simulink model "TB19_R2_Integrated_Shed"  (R2025a)
settings: Solver=FixedStepDiscrete  StartTime=0  StopTime=TB.t_end  FixedStep=TB.dt  RelTol=1e-3
InitFcn:
  | % 모델과 같은 폴더의 초기화 스크립트를 실행해 P(설계 파라미터)와 TB(시험 조건)를 만든다.
  | run(fullfile(fileparts(get_param(bdroot, 'FileName')), 'TB19_init.m'));
values from neighbouring files (symbols this model uses):
  TB = struct()    [TB19_init.m]    (also in run_TB19.m = evalin('base', 'TB'))
libraries: fl_lib x158, nesl_utility x67
(part 1 of 4)
settings Model: Creator=hj000  LastModifiedBy=hj000
settings DataIOCC: SaveOutput=off  SignalLogging=off  SaveTime=off

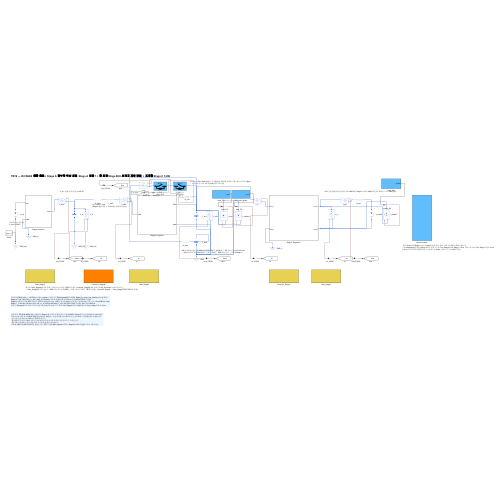
[thumbnail: Simulink's stored preview of the top-level diagram]
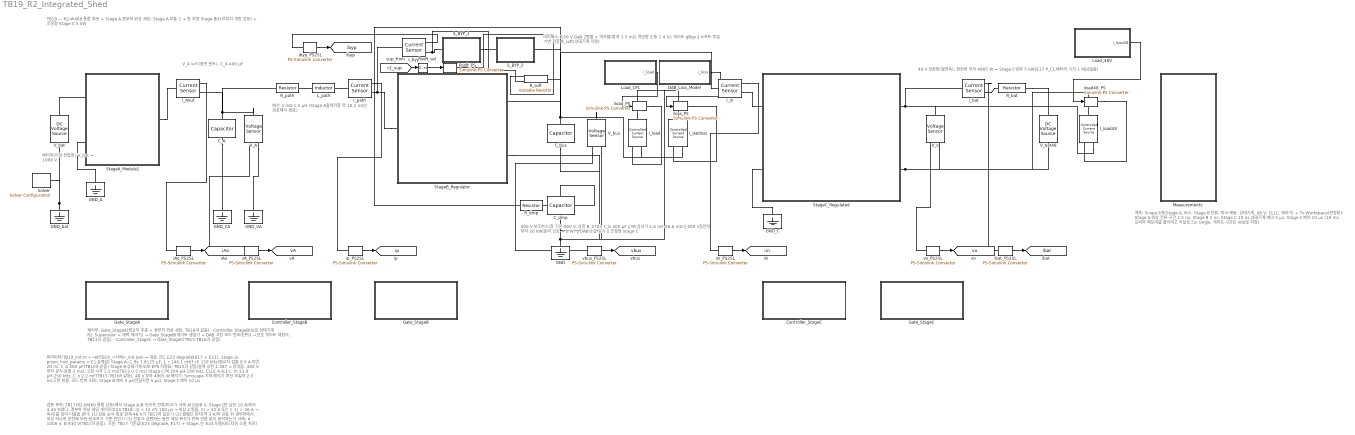
== system TB19_R2_Integrated_Shed ==
  note: TB19 — R2-W460 통합 회로 + Stage A 경부하 위상 셰딩: Stage A 모듈 1 + 창 조정 Stage B(H-브리지 개방 강등) + 조정형 Stage C 5 kW
  note: 배터리(이상 전압원)
      | V_bat = 1008 V
  note: V_A 노드(충전 포트), C_A 400 µF
  note: 배선 3 mΩ·1.5 µH
      | (Stage A 출력저항 약 10.2 mΩ는 회로에서 생김)
  note: 바이패스: 150 V GaN 2병렬 × 역직렬(합계 3.3 mΩ, 역방향 도통 1.4 V), 게이트 gByp
      | ∥ 소프트 투입 가변 저항 R_soft(상태기계 지령)
  note: 400 V 보조버스(창 기준 460 V, 상한 B_470): C_b 400 µF ∥ RC 감쇠기 1.6 mF·48.6 mΩ
      | ∥ 400 V 정전력 부하 20 kW(분리 신호 → 0 W) ∥ DAB 손실 등가 ∥ 조정형 Stage C
  note: 48 V 전원망(절연측): 정전력 부하 4905 W = Stage C 입력 5 kW(E17 P_C), 배터리 가지 1 MΩ(없음)
  note: 제어부: Gate_StageA(영교차 추종 + 경부하 위상 셰딩, TB18과 같음) · Controller_StageB(보호 상태기계 R2_Supervisor + 채택 제어기)
      | → Gate_StageB(게이트 생성기 + DAB 고장 모드 변조(EPS) → 보호 게이트 재정의, TB13과 같음) · Controller_StageC → Gate_StageC(TB15·TB16과 같음)
  note: 계측: Scope 8개(Stage A, 버스, Stage B 전류, 링크·제동, 상태기계, 48 V, CLLC, 제어기)
      | + To Workspace(판정용): Stage A 위상 전류·구간 2.5 ns, Stage B 5 ns, Stage C 10 ns, 상태기계·제어 5 µs, Stage C 제어 10 µs
      | (18 ms 모의의 메모리를 줄이려고 아날로그는 single, 게이트·구간은 int8로 저장)
  note: 파라미터(TB19_init.m ← ref/TB19_<사례>_init.json = 검증 코드 E23 degrade(E17 + E22), Stage A는 prism_hub_params = E1 설계값)
      | Stage A: C_fly 7.8125 µF, L_r 144.1 nH(f_r0 150 kHz), 영교차 검출 0.5 A·지연 20 ns, C_A 400 µF(TB16과 같음)
      | Stage B·상태기계·보호·EPS 지령표: TB13과 같음(설계 상한 1.387 × 정격점, 400 V 부하 분리·감발 3 ms). 고장 시각 1.5 ms(TB13 0.5 ms)
      | Stage C: 벅 204 µH·100 kHz, CLLC 4.8:1·L_m 33.0 µH·250 kHz, C_o 2.2 mF(TB15·TB16과 같음), 48 V 부하 4905 W
      | 해석기: Simscape 지역 해석기 후진 오일러 2.5 ns(고정 비용, 모드 반복 3회), Stage B 제어 5 µs(전달지연 5 µs), Stage C 제어 10 µs
  note: 검증 목적: TB17(R2-W460 통합 강등)에서 Stage A 끝 턴오프 전류/피크가 사례 A(1008 V, Stage C만 남은 10 A)에서 4.44 %였다.
      | 경부하 위상 셰딩 게이트(E24·TB18: |I| < 15 A가 100 µs → 위상 2 멈춤, |I| > 22 A 또는 |i_1| > 36 A → 복귀)를 넣어 다음을 본다.
      |   (1) 강등 순서·회로 한계·48 V가 TB17과 같은가
      |   (2) 클램프 유지(약 3 A)와 강등 뒤 경부하에서 위상 하나로 운전해 모든 턴오프가 기준 안인가
      |   (3) 전류가 급변하는 동안 셰딩·복귀가 반복 전환 없이 동작하는가
      | 사례: A 1008 V, B 930 V(TB17과 같음). 기준: TB17 기준값(E23 degrade, E17) + Stage A는 E24 모델(데드타임 소멸 처리)
  C_A : fl_lib/Electrical/Electrical Elements/Capacitor  c=TB.A.CA F  r=1e-6 Ohm  g=0 1/Ohm  i_specify=off  i_priority=None  i=0 A  i_nominal_specify=off  i_nominal_value=1  i_nominal_unit=A  v_specify=off  v_priority=None  v=0 V  v_nominal_specify=off  v_nominal_value=1  v_nominal_unit=V  vc_specify=on  vc_priority=High  vc=TB.vA0 V  vc_nominal_specify=off  vc_nominal_value=1  vc_nominal_unit=V
  C_bus : fl_lib/Electrical/Electrical Elements/Capacitor  c=TB.Cb F  r=1e-6 Ohm  g=0 1/Ohm  i_specify=off  i_priority=None  i=0 A  i_nominal_specify=off  i_nominal_value=1  i_nominal_unit=A  v_specify=off  v_priority=None  v=0 V  v_nominal_specify=off  v_nominal_value=1  v_nominal_unit=V  vc_specify=on  vc_priority=High  vc=TB.vb0 V  vc_nominal_specify=off  vc_nominal_value=1  vc_nominal_unit=V
  C_dmp : fl_lib/Electrical/Electrical Elements/Capacitor  c=TB.Cdmp F  r=0 Ohm  g=0 1/Ohm  i_specify=off  i_priority=None  i=0 A  i_nominal_specify=off  i_nominal_value=1  i_nominal_unit=A  v_specify=off  v_priority=None  v=0 V  v_nominal_specify=off  v_nominal_value=1  v_nominal_unit=V  vc_specify=on  vc_priority=High  vc=TB.vcd0 V  vc_nominal_specify=off  vc_nominal_value=1  vc_nominal_unit=V
  Controller_StageB : Subsystem
  Controller_StageC : Subsystem
  DAB_Loss_Model : Subsystem
  GND : fl_lib/Electrical/Electrical Elements/Electrical Reference
  GND_A : fl_lib/Electrical/Electrical Elements/Electrical Reference
  GND_C : fl_lib/Electrical/Electrical Elements/Electrical Reference
  GND_CA : fl_lib/Electrical/Electrical Elements/Electrical Reference
  GND_VA : fl_lib/Electrical/Electrical Elements/Electrical Reference
  GND_bat : fl_lib/Electrical/Electrical Elements/Electrical Reference
  Gate_StageA : Subsystem
  Gate_StageB : Subsystem
  Gate_StageC : Subsystem
  I_Aout : fl_lib/Electrical/Electrical Sensors/Current Sensor
  I_bat : fl_lib/Electrical/Electrical Sensors/Current Sensor
  I_byp : fl_lib/Electrical/Electrical Sensors/Current Sensor
  I_dabloss : fl_lib/Electrical/Electrical Sources/Controlled Current Source
  I_in : fl_lib/Electrical/Electrical Sensors/Current Sensor
  I_load : fl_lib/Electrical/Electrical Sources/Controlled Current Source
  I_load48 : fl_lib/Electrical/Electrical Sources/Controlled Current Source
  I_path : fl_lib/Electrical/Electrical Sensors/Current Sensor
  L_path : fl_lib/Electrical/Electrical Elements/Inductor  l=TB.Lpath H  r=0 Ohm  g=1e-9 1/Ohm  i_specify=off  i_priority=None  i=0 A  i_nominal_specify=off  i_nominal_value=1  i_nominal_unit=A  v_specify=off  v_priority=None  v=0 V  v_nominal_specify=off  v_nominal_value=1  v_nominal_unit=V  i_L_specify=on  i_L_priority=High  i_L=TB.ip0 A  i_L_nominal_specify=off  i_L_nominal_value=1  i_L_nominal_unit=A
  Load_48V : Subsystem
  Load_CPL : Subsystem
  Measurements : Subsystem
  R_bat : fl_lib/Electrical/Electrical Elements/Resistor  R=TB.Rbat Ohm  i_specify=off  i_priority=None  i=0 A  i_nominal_specify=off  i_nominal_value=1  i_nominal_unit=A  v_specify=off  v_priority=None  v=0 V  v_nominal_specify=off  v_nominal_value=1  v_nominal_unit=V
  R_dmp : fl_lib/Electrical/Electrical Elements/Resistor  R=TB.Rdmp Ohm  i_specify=off  i_priority=None  i=0 A  i_nominal_specify=off  i_nominal_value=1  i_nominal_unit=A  v_specify=off  v_priority=None  v=0 V  v_nominal_specify=off  v_nominal_value=1  v_nominal_unit=V
  R_path : fl_lib/Electrical/Electrical Elements/Resistor  R=TB.Rpath Ohm  i_specify=off  i_priority=None  i=0 A  i_nominal_specify=off  i_nominal_value=1  i_nominal_unit=A  v_specify=off  v_priority=None  v=0 V  v_nominal_specify=off  v_nominal_value=1  v_nominal_unit=V
  R_soft : fl_lib/Electrical/Electrical Elements/Variable Resistor  Rmin=1e-4 Ohm  thermalEnable=false  thermal_mass=1 J/K  i_specify=off  i_priority=None  i=0 A  i_nominal_specify=off  i_nominal_value=1  i_nominal_unit=A  v_specify=off  v_priority=None  v=0 V  v_nominal_specify=off  v_nominal_value=1  v_nominal_unit=V  T_specify=off  T_priority=None  T=300 K  T_nominal_specify=off  T_nominal_value=1  T_nominal_unit=K
  Rsoft_PS : nesl_utility/Simulink-PS Converter  PhysicalDomain=network_engine_domain  SubClassName=ps_input  LeftPortType=input  RightPortType=output  PseudoPeriodic=off  Frequencies=[]  NoiseDistribution=none  NoiseParameters=[]  Unit=1  AffineConversion=off  FilteringAndDerivatives=provide  SimscapeFilterOrder=1  InputFilterTimeConstant=0.001  UdotUserProvided=0
  Rsoft_sel : Selector  InputPortWidth=12  IndexOptions=Index vector (dialog)  Indices=7  OutputSizes=1
  S_BYP_1 : Subsystem  mask(PRISM-Hub switch cell){Ron=TB.Rbyp_cell, Goff=TB.B.Goff, Vf=TB.Vf_byp, Rd=TB.Rd_byp, Goffd=TB.B.Goffd}
      mask prompts: Ron "도통 저항 R_on [Ohm]"; Goff "차단 컨덕턴스 G_off [S]"; Vf "다이오드 순방향 전압 Vf [V]"; Rd "다이오드 도통 저항 R_d [Ohm]"; Goffd "다이오드 차단 컨덕턴스 [S]"
      mask help: 전력 반도체 스위치 셀 BYP1. 게이트 태그 gByp.
      settings: AttributesFormatString=gate: gByp
      mask Display:
      | plot([0.05 0.35 ],[0.50 0.50 ],[0.35 0.65 ],[0.50 0.74 ],[0.65 0.95 ],[0.50 0.50 ]);
      | plot([0.20 0.20 0.42 ],[0.50 0.20 0.20 ],[0.58 0.80 0.80 ],[0.20 0.20 0.50 ]);
      | plot([0.42 0.58 0.58 0.42 ],[0.20 0.10 0.30 0.20 ],[0.42 0.42 ],[0.10 0.30 ]);
      | text(0.5,0.80,'BYP1','horizontalAlignment','center','texmode','off');
      | port_label('LConn',1,'D');
      | port_label('RConn',1,'S');
  S_BYP_2 : Subsystem  mask(PRISM-Hub switch cell){Ron=TB.Rbyp_cell, Goff=TB.B.Goff, Vf=TB.Vf_byp, Rd=TB.Rd_byp, Goffd=TB.B.Goffd}
      mask prompts: Ron "도통 저항 R_on [Ohm]"; Goff "차단 컨덕턴스 G_off [S]"; Vf "다이오드 순방향 전압 Vf [V]"; Rd "다이오드 도통 저항 R_d [Ohm]"; Goffd "다이오드 차단 컨덕턴스 [S]"
      mask help: 전력 반도체 스위치 셀 BYP2. 게이트 태그 gByp.
      settings: AttributesFormatString=gate: gByp
      mask Display:
      | plot([0.95 0.65 ],[0.50 0.50 ],[0.65 0.35 ],[0.50 0.74 ],[0.35 0.05 ],[0.50 0.50 ]);
      | plot([0.80 0.80 0.58 ],[0.50 0.20 0.20 ],[0.42 0.20 0.20 ],[0.20 0.20 0.50 ]);
      | plot([0.58 0.42 0.42 0.58 ],[0.20 0.10 0.30 0.20 ],[0.58 0.58 ],[0.10 0.30 ]);
      | text(0.5,0.80,'BYP2','horizontalAlignment','center','texmode','off');
      | port_label('LConn',1,'D');
      | port_label('RConn',1,'S');
  Solver : nesl_utility/Solver Configuration  PhysicalDomain=network_engine_domain  SubClassName=solver  LeftPortType=input  RightPortType=generic  Tones=[]  Harmonics=[]  SimulateNoise=off  Profile=off  UseLocalSampling=off  EnableSwitchedLinearOptims=on  FrequencyDomain=off  UseCCode=off  RelTol=0.001  AbsTol=0.001  MinStep=1e-09  ToWorkspace=off  RevertToSquareIcSolve=off  NumHomotopyIterations=100  PhasorMode=off  PhasorModeNumHarmonics=1  ConsistencySolver=NEWTON_XTOL_AFTER_FTOL  IndexReductionMethod=DerivativeReplacement  DoDC=off  ResidualTolerance=1e-9  ConsistencyTolSource=GLOBAL  ConsistencyAbsTol=0.001  ConsistencyRelTol=0.001  ConsistencyTolFactor=0.001  UseLocalSolver=on  LocalSolverChoice=NE_BACKWARD_EULER_ADVANCER  ResolveIndetEquations=on  FunctionEvalNumThread=1  LocalSolverSampleTime=TB.dt  DoFixedCost=on  MaxNonlinIter=3  MaxModeIter=2  ComputeImpulses=off  ImpulseIterations=2  LinearAlgebra=auto  LinearAlgebraNumThread=0  EquationFormulation=NE_TIME_EF  DelaysMemoryBudget=1024  AutomaticFiltering=on  FilteringTimeConstant=0.001  PartitionStorageMethod=AS_NEEDED  PartitionMemoryBudget=1024  PartitionMethod=ROBUST  MultibodyUseLocalSolver=off  MultibodyLocalSolverChoice=ODE1  MultibodyLocalSolverSampleTime=0.001
  StageA_Module1 : Subsystem
  StageB_Regulator : Subsystem
  StageC_Regulated : Subsystem
  V_A : fl_lib/Electrical/Electrical Sensors/Voltage Sensor
  V_bat : fl_lib/Electrical/Electrical Sources/DC Voltage Source  v0=TB.vbat V
  V_bat48 : fl_lib/Electrical/Electrical Sources/DC Voltage Source  v0=TB.OCV V
  V_bus : fl_lib/Electrical/Electrical Sensors/Voltage Sensor
  V_o : fl_lib/Electrical/Electrical Sensors/Voltage Sensor
  iAo_PS2SL : nesl_utility/PS-Simulink Converter  PhysicalDomain=network_engine_domain  SubClassName=ps_output  LeftPortType=input  RightPortType=output  PseudoPeriodic=off  Frequencies=[]  VectorFormat=inherit  Unit=inherit  AffineConversion=off
  ibat_PS2SL : nesl_utility/PS-Simulink Converter  PhysicalDomain=network_engine_domain  SubClassName=ps_output  LeftPortType=input  RightPortType=output  PseudoPeriodic=off  Frequencies=[]  VectorFormat=inherit  Unit=inherit  AffineConversion=off
  ibyp_PS2SL : nesl_utility/PS-Simulink Converter  PhysicalDomain=network_engine_domain  SubClassName=ps_output  LeftPortType=input  RightPortType=output  PseudoPeriodic=off  Frequencies=[]  VectorFormat=inherit  Unit=inherit  AffineConversion=off
  iin_PS2SL : nesl_utility/PS-Simulink Converter  PhysicalDomain=network_engine_domain  SubClassName=ps_output  LeftPortType=input  RightPortType=output  PseudoPeriodic=off  Frequencies=[]  VectorFormat=inherit  Unit=inherit  AffineConversion=off
  iload48_PS : nesl_utility/Simulink-PS Converter  PhysicalDomain=network_engine_domain  SubClassName=ps_input  LeftPortType=input  RightPortType=output  PseudoPeriodic=off  Frequencies=[]  NoiseDistribution=none  NoiseParameters=[]  Unit=1  AffineConversion=off  FilteringAndDerivatives=provide  SimscapeFilterOrder=1  InputFilterTimeConstant=0.001  UdotUserProvided=0
  iload_PS : nesl_utility/Simulink-PS Converter  PhysicalDomain=network_engine_domain  SubClassName=ps_input  LeftPortType=input  RightPortType=output  PseudoPeriodic=off  Frequencies=[]  NoiseDistribution=none  NoiseParameters=[]  Unit=1  AffineConversion=off  FilteringAndDerivatives=provide  SimscapeFilterOrder=1  InputFilterTimeConstant=0.001  UdotUserProvided=0
  iloss_PS : nesl_utility/Simulink-PS Converter  PhysicalDomain=network_engine_domain  SubClassName=ps_input  LeftPortType=input  RightPortType=output  PseudoPeriodic=off  Frequencies=[]  NoiseDistribution=none  NoiseParameters=[]  Unit=1  AffineConversion=off  FilteringAndDerivatives=provide  SimscapeFilterOrder=1  InputFilterTimeConstant=0.001  UdotUserProvided=0
  ip_PS2SL : nesl_utility/PS-Simulink Converter  PhysicalDomain=network_engine_domain  SubClassName=ps_output  LeftPortType=input  RightPortType=output  PseudoPeriodic=off  Frequencies=[]  VectorFormat=inherit  Unit=inherit  AffineConversion=off
  vA_PS2SL : nesl_utility/PS-Simulink Converter  PhysicalDomain=network_engine_domain  SubClassName=ps_output  LeftPortType=input  RightPortType=output  PseudoPeriodic=off  Frequencies=[]  VectorFormat=inherit  Unit=inherit  AffineConversion=off
  vbus_PS2SL : nesl_utility/PS-Simulink Converter  PhysicalDomain=network_engine_domain  SubClassName=ps_output  LeftPortType=input  RightPortType=output  PseudoPeriodic=off  Frequencies=[]  VectorFormat=inherit  Unit=inherit  AffineConversion=off
  vo_PS2SL : nesl_utility/PS-Simulink Converter  PhysicalDomain=network_engine_domain  SubClassName=ps_output  LeftPortType=input  RightPortType=output  PseudoPeriodic=off  Frequencies=[]  VectorFormat=inherit  Unit=inherit  AffineConversion=off
  tag scope: iAo=global, ibat=global, ibyp=global, iin=global, ip=global, vA=global, vbus=global, vo=global
  wires:
  iAo_PS2SL/1 -> [iAo]
  vA_PS2SL/1 -> [vA]
  [r2_sup] -> Rsoft_sel/1
  Rsoft_sel/1 -> Rsoft_PS/1
  ip_PS2SL/1 -> [ip]
  vbus_PS2SL/1 -> [vbus]
  ibyp_PS2SL/1 -> [ibyp]
  Load_CPL/1(i_load) -> iload_PS/1
  DAB_Loss_Model/1(i_loss) -> iloss_PS/1
  iin_PS2SL/1 -> [iin]
  vo_PS2SL/1 -> [vo]
  ibat_PS2SL/1 -> [ibat]
  Load_48V/1(i_load48) -> iload48_PS/1
  connections:
  GND_bat/LConn1 -- Solver/RConn1 -- V_bat/RConn1
  V_bat/LConn1 -- StageA_Module1/LConn1
  StageA_Module1/LConn2 -- GND_A/LConn1
  StageA_Module1/RConn1 -- I_Aout/LConn1
  I_Aout/RConn2 -- V_A/LConn1 -- C_A/LConn1 -- R_path/LConn1
  C_A/RConn1 -- GND_CA/LConn1
  V_A/RConn2 -- GND_VA/LConn1
  R_path/RConn1 -- L_path/LConn1
  L_path/RConn1 -- I_path/LConn1
  I_Aout/RConn1 -- iAo_PS2SL/LConn1
  V_A/RConn1 -- vA_PS2SL/LConn1
  StageB_Regulator/LConn1 -- I_path/RConn2 -- I_byp/LConn1
  S_BYP_1/LConn1 -- I_byp/RConn2 -- R_soft/LConn2
  S_BYP_1/RConn1 -- S_BYP_2/RConn1
  S_BYP_2/LConn1 -- R_soft/RConn1 -- StageB_Regulator/RConn1 -- R_dmp/LConn1 -- V_bus/LConn1 -- I_load/RConn2 -- I_dabloss/RConn2 -- C_bus/LConn1 -- I_in/LConn1
  Rsoft_PS/RConn1 -- R_soft/LConn1
  StageB_Regulator/RConn2 -- C_bus/RConn1 -- C_dmp/RConn1 -- V_bus/RConn2 -- I_load/LConn1 -- GND/LConn1 -- I_dabloss/LConn1
  R_dmp/RConn1 -- C_dmp/LConn1
  iload_PS/RConn1 -- I_load/RConn1
  iloss_PS/RConn1 -- I_dabloss/RConn1
  I_path/RConn1 -- ip_PS2SL/LConn1
  V_bus/RConn1 -- vbus_PS2SL/LConn1
  I_byp/RConn1 -- ibyp_PS2SL/LConn1
  I_in/RConn2 -- StageC_Regulated/LConn1
  StageC_Regulated/LConn2 -- GND_C/LConn1
  V_o/LConn1 -- I_bat/LConn1 -- StageC_Regulated/RConn1 -- I_load48/RConn2
  V_o/RConn2 -- V_bat48/RConn1 -- StageC_Regulated/RConn2 -- I_load48/LConn1
  I_bat/RConn2 -- R_bat/LConn1
  R_bat/RConn1 -- V_bat48/LConn1
  iload48_PS/RConn1 -- I_load48/RConn1
  I_in/RConn1 -- iin_PS2SL/LConn1
  V_o/RConn1 -- vo_PS2SL/LConn1
  I_bat/RConn1 -- ibat_PS2SL/LConn1

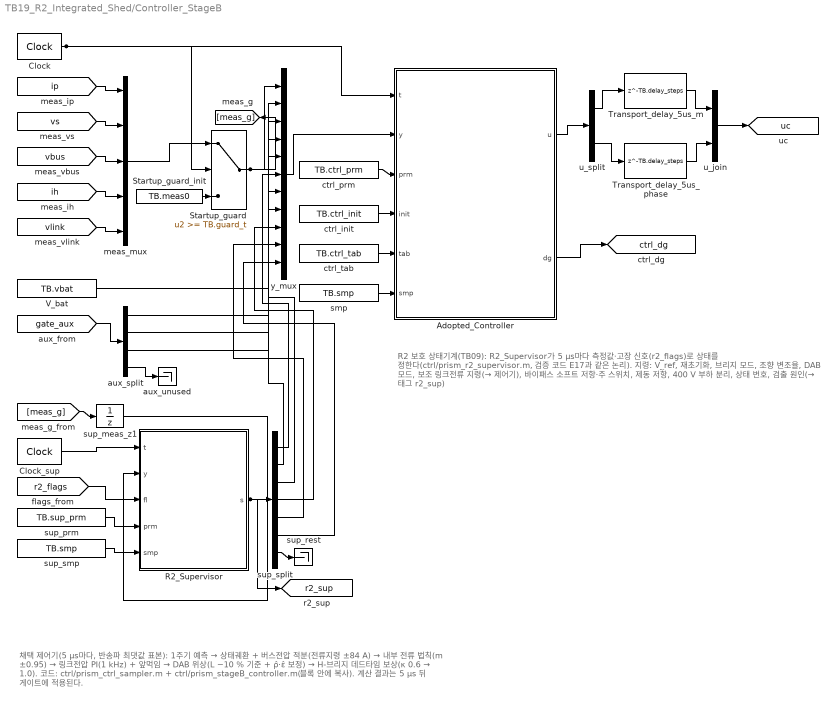
== system TB19_R2_Integrated_Shed/Controller_StageB ==
  note: R2 보호 상태기계(TB09): R2_Supervisor가 5 µs마다 측정값·고장 신호(r2_flags)로 상태를 정한다(ctrl/prism_r2_supervisor.m,
      | 검증 코드 E17과 같은 논리). 지령: V_ref, 재초기화, 브리지 모드, 조향 변조율, DAB 모드, 보조 링크전류 지령(→ 제어기),
      | 바이패스 소프트 저항·주 스위치, 제동 저항, 400 V 부하 분리, 상태 번호, 검출 원인(→ 태그 r2_sup)
  note: 채택 제어기(5 µs마다, 반송파 최댓값 표본): 1주기 예측 → 상태궤환 + 버스전압 적분(전류지령 ±84 A) → 내부 전류 법칙(m ±0.95)
      | → 링크전압 PI(1 kHz) + 앞먹임 → DAB 위상(L −10 % 기준 + ρ̂·ε̂ 보정) → H-브리지 데드타임 보상(κ 0.6 → 1.0).
      | 코드: ctrl/prism_ctrl_sampler.m + ctrl/prism_stageB_controller.m(블록 안에 복사). 계산 결과는 5 µs 뒤 게이트에 적용된다.
  Adopted_Controller : MATLAB Function  TreatAsAtomicUnit=on
  Clock : DigitalClock  SampleTime=TB.dt
  Clock_sup : DigitalClock  SampleTime=TB.dt
  R2_Supervisor : MATLAB Function  TreatAsAtomicUnit=on
  Startup_guard : Switch  Threshold=TB.guard_t  SaturateOnIntegerOverflow=off  InputSameDT=off
  Startup_guard_init : Constant  Value=TB.meas0
  Transport_delay_5us_m : Delay  DelayLength=TB.delay_steps  InitialCondition=TB.uc0(1)
  Transport_delay_5us_phase : Delay  DelayLength=TB.delay_steps  InitialCondition=TB.uc0(2)
  V_bat : Constant  Value=TB.vbat
  aux_split : Demux  Outputs=[1 1 1 3]
  aux_unused : Terminator
  ctrl_init : Constant  Value=TB.ctrl_init
  ctrl_prm : Constant  Value=TB.ctrl_prm
  ctrl_tab : Constant  Value=TB.ctrl_tab
  meas_mux : Mux  Inputs=5
  smp : Constant  Value=TB.smp
  sup_meas_z1 : UnitDelay  InitialCondition=TB.meas0'  SampleTime=TB.dt  HasFrameUpgradeWarning=on
  sup_prm : Constant  Value=TB.sup_prm
  sup_rest : Terminator
  sup_smp : Constant  Value=TB.smp
  sup_split : Demux  Outputs=[1 1 1 1 1 1 6]
  u_join : Mux  Inputs=2
  u_split : Demux  Outputs=2
  y_mux : Mux  Inputs=11
  tag scope: ctrl_dg=global, r2_sup=global, uc=global
  wires:
  [ip] -> meas_mux/1
  [vs] -> meas_mux/2
  [vbus] -> meas_mux/3
  [ih] -> meas_mux/4
  [vlink] -> meas_mux/5
  Startup_guard_init/1 -> Startup_guard/3
  meas_mux/1 -> Startup_guard/1
  Clock/1 -> Startup_guard/2, Adopted_Controller/1(t)
  Startup_guard/1 -> y_mux/1, [meas_g]
  V_bat/1 -> y_mux/2
  [gate_aux] -> aux_split/1
  aux_split/1 -> y_mux/3
  aux_split/2 -> y_mux/4
  aux_split/3 -> y_mux/5
  aux_split/4 -> aux_unused/1
  Clock_sup/1 -> R2_Supervisor/1(t)
  [meas_g] -> sup_meas_z1/1
  sup_meas_z1/1 -> R2_Supervisor/2(y)
  [r2_flags] -> R2_Supervisor/3(fl)
  sup_prm/1 -> R2_Supervisor/4(prm)
  sup_smp/1 -> R2_Supervisor/5(smp)
  R2_Supervisor/1(s) -> [r2_sup], sup_split/1
  sup_split/1 -> y_mux/6
  sup_split/2 -> y_mux/7
  sup_split/3 -> y_mux/8
  sup_split/4 -> y_mux/9
  sup_split/5 -> y_mux/10
  sup_split/6 -> y_mux/11
  sup_split/7 -> sup_rest/1
  y_mux/1 -> Adopted_Controller/2(y)
  ctrl_prm/1 -> Adopted_Controller/3(prm)
  ctrl_init/1 -> Adopted_Controller/4(init)
  ctrl_tab/1 -> Adopted_Controller/5(tab)
  smp/1 -> Adopted_Controller/6(smp)
  Adopted_Controller/1(u) -> u_split/1
  u_split/1 -> Transport_delay_5us_m/1
  u_split/2 -> Transport_delay_5us_phase/1
  Transport_delay_5us_m/1 -> u_join/1
  Transport_delay_5us_phase/1 -> u_join/2
  u_join/1 -> [uc]
  Adopted_Controller/2(dg) -> [ctrl_dg]

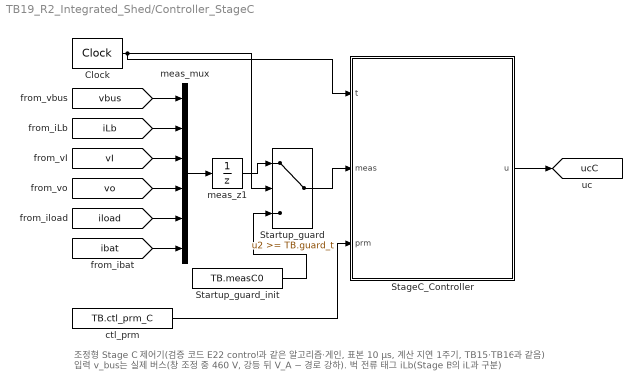
== system TB19_R2_Integrated_Shed/Controller_StageC ==
  note: 조정형 Stage C 제어기(검증 코드 E22 control과 같은 알고리즘·게인, 표본 10 µs, 계산 지연 1주기, TB15·TB16과 같음)
      | 입력 v_bus는 실제 버스(창 조정 중 460 V, 강등 뒤 V_A − 경로 강하). 벅 전류 태그 iLb(Stage B의 iL과 구분)
  Clock : DigitalClock  SampleTime=TB.dt
  StageC_Controller : MATLAB Function  TreatAsAtomicUnit=on
  Startup_guard : Switch  Threshold=TB.guard_t  SaturateOnIntegerOverflow=off  InputSameDT=off
  Startup_guard_init : Constant  Value=TB.measC0
  ctl_prm : Constant  Value=TB.ctl_prm_C
  meas_mux : Mux  Inputs=6
  meas_z1 : UnitDelay  InitialCondition=TB.measC0  SampleTime=TB.dt  HasFrameUpgradeWarning=on
  tag scope: ucC=global
  wires:
  [vbus] -> meas_mux/1
  [iLb] -> meas_mux/2
  [vI] -> meas_mux/3
  [vo] -> meas_mux/4
  [iload] -> meas_mux/5
  [ibat] -> meas_mux/6
  meas_mux/1 -> meas_z1/1
  Startup_guard_init/1 -> Startup_guard/3
  meas_z1/1 -> Startup_guard/1
  Clock/1 -> Startup_guard/2, StageC_Controller/1(t)
  Startup_guard/1 -> StageC_Controller/2(meas)
  ctl_prm/1 -> StageC_Controller/3(prm)
  StageC_Controller/1(u) -> [ucC]

== system TB19_R2_Integrated_Shed/DAB_Loss_Model ==
  note: DAB 손실 등가: 직전 주기 평균 링크전력 p̄로 P_loss = (1/η − 1)max(p̄,0) + (1 − η)max(−p̄,0) − R_dab·mean(i_L²)
      | (η = 0.96, 검증 모델과 같음)을 버스 전류 P_loss/v_bus로 끈다. 회로의 R_dab 손실은 빼서 중복을 막는다.
  Clock : DigitalClock  SampleTime=TB.dt
  DAB_Loss : MATLAB Function  TreatAsAtomicUnit=on
  Startup_guard : Switch  Threshold=TB.guard_t  SaturateOnIntegerOverflow=off  InputSameDT=off
  Startup_guard_init : Constant  Value=TB.loss_meas0
  iloss_z1 : UnitDelay  SampleTime=TB.dt  HasFrameUpgradeWarning=on
  loss_prm : Constant  Value=TB.loss_prm
  meas_mux : Mux
  meas_split : Demux
  ploss0 : Constant  Value=TB.ploss0
  i_loss : Outport
  wires:
  [vlink] -> meas_mux/1
  [ilink] -> meas_mux/2
  [iL] -> meas_mux/3
  [vbus] -> meas_mux/4
  Startup_guard_init/1 -> Startup_guard/3
  meas_mux/1 -> Startup_guard/1
  Clock/1 -> Startup_guard/2, DAB_Loss/1(t)
  Startup_guard/1 -> meas_split/1
  meas_split/1 -> DAB_Loss/2(vl)
  meas_split/2 -> DAB_Loss/3(il)
  meas_split/3 -> DAB_Loss/4(iL)
  meas_split/4 -> DAB_Loss/5(vb)
  loss_prm/1 -> DAB_Loss/6(prm)
  ploss0/1 -> DAB_Loss/7(ploss0)
  DAB_Loss/1(iloss) -> iloss_z1/1
  iloss_z1/1 -> i_loss/1

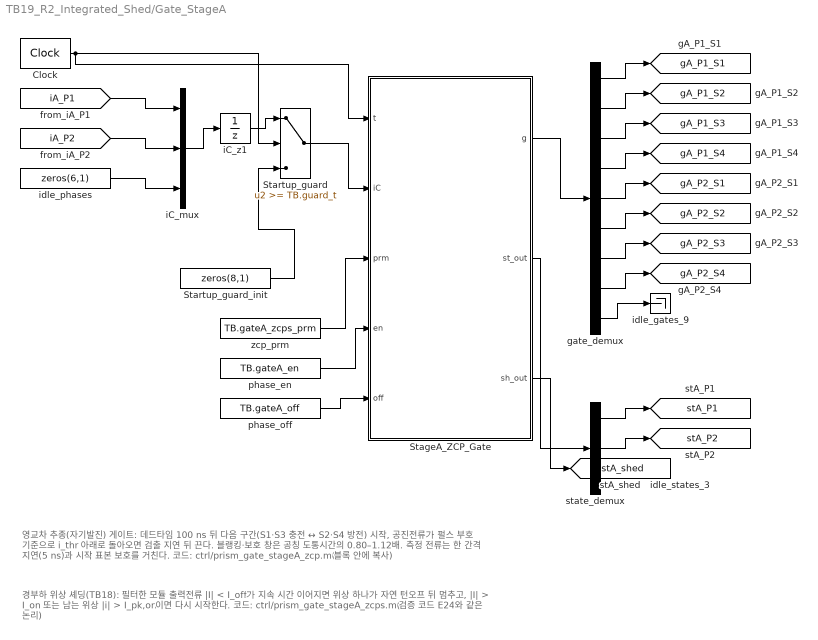
== system TB19_R2_Integrated_Shed/Gate_StageA ==
  note: 경부하 위상 셰딩(TB18): 필터한 모듈 출력전류 |I| < I_off가 지속 시간 이어지면 위상 하나가 자연 턴오프 뒤 멈추고,
      | |I| > I_on 또는 남는 위상 |i| > I_pk,on이면 다시 시작한다. 코드: ctrl/prism_gate_stageA_zcps.m(검증 코드 E24와 같은 논리)
  note: 영교차 추종(자기발진) 게이트: 데드타임 100 ns 뒤 다음 구간(S1·S3 충전 ↔ S2·S4 방전) 시작,
      | 공진전류가 펄스 부호 기준으로 i_thr 아래로 돌아오면 검출 지연 뒤 끈다. 블랭킹·보호 창은 공칭 도통시간의 0.80–1.12배.
      | 측정 전류는 한 간격 지연(5 ns)과 시작 표본 보호를 거친다. 코드: ctrl/prism_gate_stageA_zcp.m(블록 안에 복사)
  Clock : DigitalClock  SampleTime=TB.dt
  StageA_ZCP_Gate : MATLAB Function  TreatAsAtomicUnit=on
  Startup_guard : Switch  Threshold=TB.guard_t  SaturateOnIntegerOverflow=off  InputSameDT=off
  Startup_guard_init : Constant  Value=zeros(8,1)
  gate_demux : Demux  Outputs=[1 1 1 1 1 1 1 1 24]
  iC_mux : Mux  Inputs=3
  iC_z1 : UnitDelay  SampleTime=TB.dt  HasFrameUpgradeWarning=on
  idle_gates_9 : Terminator
  idle_phases : Constant  Value=zeros(6,1)
  idle_states_3 : Terminator
  phase_en : Constant  Value=TB.gateA_en
  phase_off : Constant  Value=TB.gateA_off
  state_demux : Demux  Outputs=[1 1 6]
  zcp_prm : Constant  Value=TB.gateA_zcps_prm
  tag scope: gA_P1_S1=global, gA_P1_S2=global, gA_P1_S3=global, gA_P1_S4=global, gA_P2_S1=global, gA_P2_S2=global, gA_P2_S3=global, gA_P2_S4=global, stA_P1=global, stA_P2=global, stA_shed=global
  wires:
  [iA_P1] -> iC_mux/1
  [iA_P2] -> iC_mux/2
  idle_phases/1 -> iC_mux/3
  iC_mux/1 -> iC_z1/1
  Startup_guard_init/1 -> Startup_guard/3
  iC_z1/1 -> Startup_guard/1
  Clock/1 -> Startup_guard/2, StageA_ZCP_Gate/1(t)
  StageA_ZCP_Gate/3(sh_out) -> [stA_shed]
  Startup_guard/1 -> StageA_ZCP_Gate/2(iC)
  zcp_prm/1 -> StageA_ZCP_Gate/3(prm)
  phase_en/1 -> StageA_ZCP_Gate/4(en)
  phase_off/1 -> StageA_ZCP_Gate/5(off)
  StageA_ZCP_Gate/1(g) -> gate_demux/1
  gate_demux/1 -> [gA_P1_S1]
  gate_demux/2 -> [gA_P1_S2]
  gate_demux/3 -> [gA_P1_S3]
  gate_demux/4 -> [gA_P1_S4]
  gate_demux/5 -> [gA_P2_S1]
  gate_demux/6 -> [gA_P2_S2]
  gate_demux/7 -> [gA_P2_S3]
  gate_demux/8 -> [gA_P2_S4]
  gate_demux/9 -> idle_gates_9/1
  StageA_ZCP_Gate/2(st_out) -> state_demux/1
  state_demux/1 -> [stA_P1]
  state_demux/2 -> [stA_P2]
  state_demux/3 -> idle_states_3/1

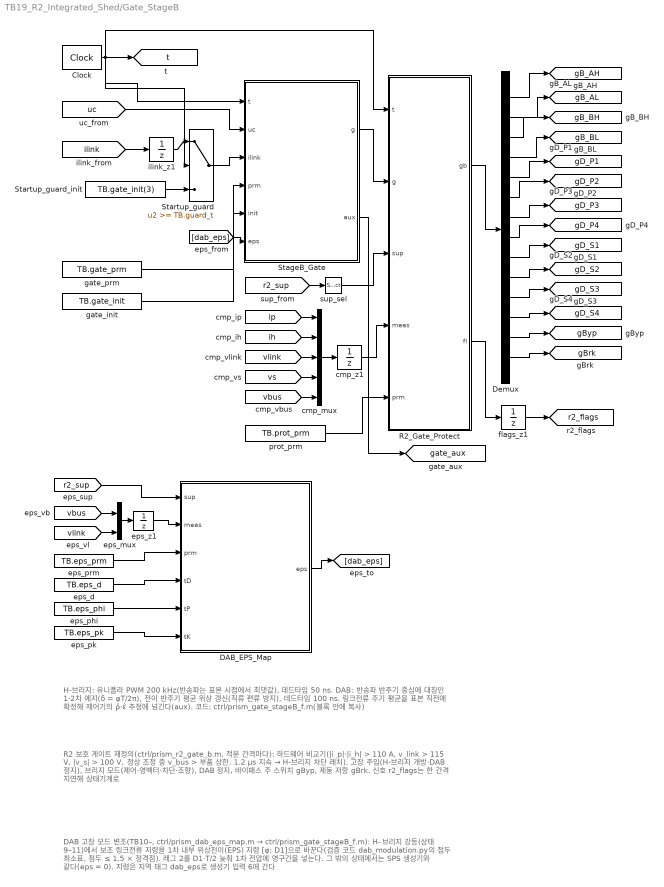
== system TB19_R2_Integrated_Shed/Gate_StageB ==
  note: H-브리지: 유니폴라 PWM 200 kHz(반송파는 표본 시점에서 최댓값), 데드타임 50 ns.
      | DAB: 반송파 반주기 중심에 대칭인 1·2차 에지(δ = φT/2π), 전이 반주기 평균 위상 갱신(직류 편류 방지), 데드타임 100 ns.
      | 링크전류 주기 평균을 표본 직전에 확정해 제어기의 ρ̂·ε̂ 추정에 넘긴다(aux). 코드: ctrl/prism_gate_stageB_f.m(블록 안에 복사)
  note: DAB 고장 모드 변조(TB10–, ctrl/prism_dab_eps_map.m → ctrl/prism_gate_stageB_f.m): H-브리지 강등(상태 9–11)에서 보조 링크전류 지령을
      | 1차 내부 위상천이(EPS) 지령 [φ; D1]으로 바꾼다(검증 코드 dab_modulation.py의 첨두 최소표, 첨두 ≤ 1.5 × 정격점). 레그 2를 D1·T/2 늦춰
      | 1차 전압에 영구간을 넣는다. 그 밖의 상태에서는 SPS 생성기와 같다(eps = 0). 지령은 지역 태그 dab_eps로 생성기 입력 6에 간다
  note: R2 보호 게이트 재정의(ctrl/prism_r2_gate_b.m, 적분 간격마다): 하드웨어 비교기(|i_p|·|i_h| > 110 A, v_link > 115 V,
      | |v_s| > 100 V, 정상 조정 중 v_bus > 부품 상한, 1.2 µs 지속 → H-브리지 차단 래치), 고장 주입(H-브리지 개방·DAB 정지),
      | 브리지 모드(제어·영벡터·차단·조향), DAB 정지, 바이패스 주 스위치 gByp, 제동 저항 gBrk. 신호 r2_flags는 한 간격 지연해 상태기계로
  Clock : DigitalClock  SampleTime=TB.dt
  DAB_EPS_Map : MATLAB Function  TreatAsAtomicUnit=on
  Demux : Demux  Outputs=14
  R2_Gate_Protect : MATLAB Function  TreatAsAtomicUnit=on
  StageB_Gate : MATLAB Function  TreatAsAtomicUnit=on
  Startup_guard : Switch  Threshold=TB.guard_t  SaturateOnIntegerOverflow=off  InputSameDT=off
  Startup_guard_init : Constant  Value=TB.gate_init(3)
  cmp_mux : Mux  Inputs=5
  cmp_z1 : UnitDelay  InitialCondition=[TB.ip0 TB.ih0 TB.vl0 TB.vs0 TB.vb0]'  SampleTime=TB.dt  HasFrameUpgradeWarning=on
  eps_d : Constant  Value=TB.eps_d
  eps_mux : Mux  Inputs=2
  eps_phi : Constant  Value=TB.eps_phi
  eps_pk : Constant  Value=TB.eps_pk
  eps_prm : Constant  Value=TB.eps_prm
  eps_z1 : UnitDelay  InitialCondition=[TB.vb0 TB.vl0]'  SampleTime=TB.dt  HasFrameUpgradeWarning=on
  flags_z1 : UnitDelay  SampleTime=TB.dt  HasFrameUpgradeWarning=on
  gate_init : Constant  Value=TB.gate_init
  gate_prm : Constant  Value=TB.gate_prm
  ilink_z1 : UnitDelay  SampleTime=TB.dt  HasFrameUpgradeWarning=on
  prot_prm : Constant  Value=TB.prot_prm
  sup_sel : Selector  InputPortWidth=12  IndexOptions=Index vector (dialog)  Indices=[3 5 8 9 11]  OutputSizes=1
  tag scope: gB_AH=global, gB_AL=global, gB_BH=global, gB_BL=global, gBrk=global, gByp=global, gD_P1=global, gD_P2=global, gD_P3=global, gD_P4=global, gD_S1=global, gD_S2=global, gD_S3=global, gD_S4=global, gate_aux=global, r2_flags=global, t=global
  wires:
  Startup_guard_init/1 -> Startup_guard/3
  Clock/1 -> [t], StageB_Gate/1(t), Startup_guard/2, R2_Gate_Protect/1(t)
  [uc] -> StageB_Gate/2(uc)
  [ilink] -> ilink_z1/1
  ilink_z1/1 -> Startup_guard/1
  Startup_guard/1 -> StageB_Gate/3(ilink)
  gate_prm/1 -> StageB_Gate/4(prm)
  gate_init/1 -> StageB_Gate/5(init)
  [r2_sup] -> sup_sel/1
  [ip] -> cmp_mux/1
  [ih] -> cmp_mux/2
  [vlink] -> cmp_mux/3
  [vs] -> cmp_mux/4
  [vbus] -> cmp_mux/5
  cmp_mux/1 -> cmp_z1/1
  StageB_Gate/1(g) -> R2_Gate_Protect/2(g)
  sup_sel/1 -> R2_Gate_Protect/3(sup)
  cmp_z1/1 -> R2_Gate_Protect/4(meas)
  prot_prm/1 -> R2_Gate_Protect/5(prm)
  R2_Gate_Protect/1(gb) -> Demux/1
  R2_Gate_Protect/2(fl) -> flags_z1/1
  flags_z1/1 -> [r2_flags]
  [vbus] -> eps_mux/1
  [vlink] -> eps_mux/2
  eps_mux/1 -> eps_z1/1
  [r2_sup] -> DAB_EPS_Map/1(sup)
  eps_z1/1 -> DAB_EPS_Map/2(meas)
  eps_prm/1 -> DAB_EPS_Map/3(prm)
  eps_d/1 -> DAB_EPS_Map/4(tD)
  eps_phi/1 -> DAB_EPS_Map/5(tP)
  eps_pk/1 -> DAB_EPS_Map/6(tK)
  DAB_EPS_Map/1(eps) -> [dab_eps]
  [dab_eps] -> StageB_Gate/6(eps)
  Demux/1 -> [gB_AH]
  Demux/2 -> [gB_AL]
  Demux/3 -> [gB_BH]
  Demux/4 -> [gB_BL]
  Demux/5 -> [gD_P1]
  Demux/6 -> [gD_P2]
  Demux/7 -> [gD_P3]
  Demux/8 -> [gD_P4]
  Demux/9 -> [gD_S1]
  Demux/10 -> [gD_S2]
  Demux/11 -> [gD_S3]
  Demux/12 -> [gD_S4]
  Demux/13 -> [gByp]
  Demux/14 -> [gBrk]
  StageB_Gate/2(aux) -> [gate_aux]

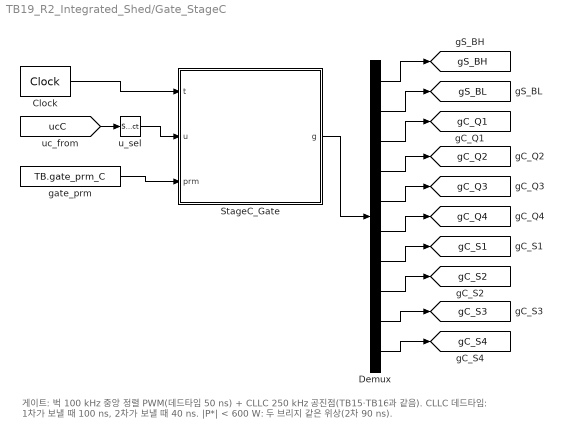
== system TB19_R2_Integrated_Shed/Gate_StageC ==
  note: 게이트: 벅 100 kHz 중앙 정렬 PWM(데드타임 50 ns) + CLLC 250 kHz 공진점(TB15·TB16과 같음).
      | CLLC 데드타임: 1차가 보낼 때 100 ns, 2차가 보낼 때 40 ns. |P*| < 600 W: 두 브리지 같은 위상(2차 90 ns).
  Clock : DigitalClock  SampleTime=TB.dt
  Demux : Demux  Outputs=10
  StageC_Gate : MATLAB Function  TreatAsAtomicUnit=on
  gate_prm : Constant  Value=TB.gate_prm_C
  u_sel : Selector  InputPortWidth=4  IndexOptions=Index vector (dialog)  Indices=[1 2]  OutputSizes=1
  tag scope: gC_Q1=global, gC_Q2=global, gC_Q3=global, gC_Q4=global, gC_S1=global, gC_S2=global, gC_S3=global, gC_S4=global, gS_BH=global, gS_BL=global
  wires:
  [ucC] -> u_sel/1
  Clock/1 -> StageC_Gate/1(t)
  u_sel/1 -> StageC_Gate/2(u)
  gate_prm/1 -> StageC_Gate/3(prm)
  StageC_Gate/1(g) -> Demux/1
  Demux/1 -> [gS_BH]
  Demux/2 -> [gS_BL]
  Demux/3 -> [gC_Q1]
  Demux/4 -> [gC_Q2]
  Demux/5 -> [gC_Q3]
  Demux/6 -> [gC_Q4]
  Demux/7 -> [gC_S1]
  Demux/8 -> [gC_S2]
  Demux/9 -> [gC_S3]
  Demux/10 -> [gC_S4]

== system TB19_R2_Integrated_Shed/Load_48V ==
  note: 48 V 정전력 부하(시험 장치): i = P48/max(v_o, 10 V). v_o는 시작 표본 보호 후 한 간격 지연(대수 루프 방지)
  Guard_vo : Switch  Threshold=TB.guard_t  SaturateOnIntegerOverflow=off  InputSameDT=off
  Guard_vo_init : Constant  Value=TB.x0(3)
  P48 : Constant  Value=TB.P48
  P_over_v : Product  Inputs=*/
  v_floor : MinMax  Function=max  Inputs=2
  v_min : Constant  Value=TB.vmin_cpl
  vo_z1 : UnitDelay  SampleTime=TB.dt  HasFrameUpgradeWarning=on
  i_load48 : Outport
  tag scope: iload=global, p48=global
  wires:
  Guard_vo_init/1 -> Guard_vo/3
  P48/1 -> [p48], P_over_v/1
  [vo] -> Guard_vo/1
  [t] -> Guard_vo/2
  Guard_vo/1 -> vo_z1/1
  vo_z1/1 -> v_floor/1
  v_min/1 -> v_floor/2
  v_floor/1 -> P_over_v/2
  P_over_v/1 -> [iload], i_load48/1

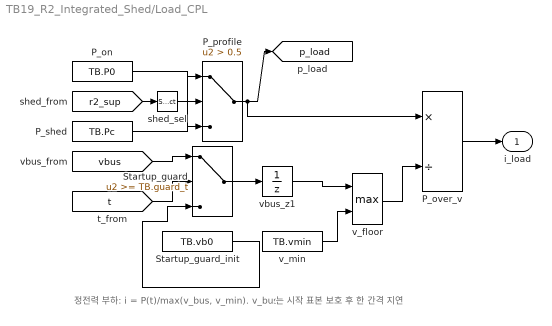
== system TB19_R2_Integrated_Shed/Load_CPL ==
  note: 정전력 부하: i = P(t)/max(v_bus, v_min). v_bus는 시작 표본 보호 후 한 간격 지연
  P_on : Constant  Value=TB.P0
  P_over_v : Product  Inputs=*/
  P_profile : Switch  Criteria=u2 > Threshold  Threshold=0.5  SaturateOnIntegerOverflow=off  InputSameDT=off
  P_shed : Constant  Value=TB.Pc
  Startup_guard : Switch  Threshold=TB.guard_t  SaturateOnIntegerOverflow=off  InputSameDT=off
  Startup_guard_init : Constant  Value=TB.vb0
  shed_sel : Selector  InputPortWidth=12  IndexOptions=Index vector (dialog)  Indices=10  OutputSizes=1
  v_floor : MinMax  Function=max  Inputs=2
  v_min : Constant  Value=TB.vmin
  vbus_z1 : UnitDelay  SampleTime=TB.dt  HasFrameUpgradeWarning=on
  i_load : Outport
  tag scope: p_load=global
  wires:
  P_shed/1 -> P_profile/1
  [r2_sup] -> shed_sel/1
  shed_sel/1 -> P_profile/2
  P_on/1 -> P_profile/3
  Startup_guard_init/1 -> Startup_guard/3
  P_profile/1 -> [p_load], P_over_v/1
  [vbus] -> Startup_guard/1
  [t] -> Startup_guard/2
  Startup_guard/1 -> vbus_z1/1
  vbus_z1/1 -> v_floor/1
  v_min/1 -> v_floor/2
  v_floor/1 -> P_over_v/2
  P_over_v/1 -> i_load/1

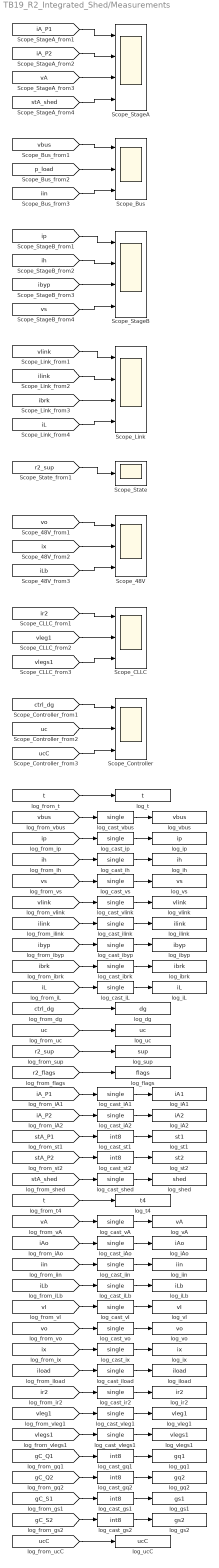
== system TB19_R2_Integrated_Shed/Measurements ==
  Scope_48V : Scope  NumInputPorts=3
      settings: Title=Scope 48V
  Scope_Bus : Scope  NumInputPorts=3
      settings: Title=Scope Bus
  Scope_CLLC : Scope  NumInputPorts=3
      settings: Title=Scope CLLC
  Scope_Controller : Scope  NumInputPorts=3
      settings: Title=Scope Controller
  Scope_Link : Scope  NumInputPorts=4
      settings: Title=Scope Link
  Scope_StageA : Scope  NumInputPorts=4
      settings: Title=Scope StageA
  Scope_StageB : Scope  NumInputPorts=4
      settings: Title=Scope StageB
  Scope_State : Scope
      settings: Title=Scope State
  log_cast_gq1 : DataTypeConversion  OutDataTypeStr=int8  SaturateOnIntegerOverflow=off  RndMeth=Floor
  log_cast_gq2 : DataTypeConversion  OutDataTypeStr=int8  SaturateOnIntegerOverflow=off  RndMeth=Floor
  log_cast_gs1 : DataTypeConversion  OutDataTypeStr=int8  SaturateOnIntegerOverflow=off  RndMeth=Floor
  log_cast_gs2 : DataTypeConversion  OutDataTypeStr=int8  SaturateOnIntegerOverflow=off  RndMeth=Floor
  log_cast_iA1 : DataTypeConversion  OutDataTypeStr=single  SaturateOnIntegerOverflow=off  RndMeth=Floor
  log_cast_iA2 : DataTypeConversion  OutDataTypeStr=single  SaturateOnIntegerOverflow=off  RndMeth=Floor
  log_cast_iAo : DataTypeConversion  OutDataTypeStr=single  SaturateOnIntegerOverflow=off  RndMeth=Floor
  log_cast_iL : DataTypeConversion  OutDataTypeStr=single  SaturateOnIntegerOverflow=off  RndMeth=Floor
  log_cast_iLb : DataTypeConversion  OutDataTypeStr=single  SaturateOnIntegerOverflow=off  RndMeth=Floor
  log_cast_ibrk : DataTypeConversion  OutDataTypeStr=single  SaturateOnIntegerOverflow=off  RndMeth=Floor
  log_cast_ibyp : DataTypeConversion  OutDataTypeStr=single  SaturateOnIntegerOverflow=off  RndMeth=Floor
  log_cast_ih : DataTypeConversion  OutDataTypeStr=single  SaturateOnIntegerOverflow=off  RndMeth=Floor
  log_cast_iin : DataTypeConversion  OutDataTypeStr=single  SaturateOnIntegerOverflow=off  RndMeth=Floor
  log_cast_ilink : DataTypeConversion  OutDataTypeStr=single  SaturateOnIntegerOverflow=off  RndMeth=Floor
  log_cast_iload : DataTypeConversion  OutDataTypeStr=single  SaturateOnIntegerOverflow=off  RndMeth=Floor
  log_cast_ip : DataTypeConversion  OutDataTypeStr=single  SaturateOnIntegerOverflow=off  RndMeth=Floor
  log_cast_ir2 : DataTypeConversion  OutDataTypeStr=single  SaturateOnIntegerOverflow=off  RndMeth=Floor
  log_cast_ix : DataTypeConversion  OutDataTypeStr=single  SaturateOnIntegerOverflow=off  RndMeth=Floor
  log_cast_shed : DataTypeConversion  OutDataTypeStr=single  SaturateOnIntegerOverflow=off  RndMeth=Floor
  log_cast_st1 : DataTypeConversion  OutDataTypeStr=int8  SaturateOnIntegerOverflow=off  RndMeth=Floor
  log_cast_st2 : DataTypeConversion  OutDataTypeStr=int8  SaturateOnIntegerOverflow=off  RndMeth=Floor
  log_cast_vA : DataTypeConversion  OutDataTypeStr=single  SaturateOnIntegerOverflow=off  RndMeth=Floor
  log_cast_vI : DataTypeConversion  OutDataTypeStr=single  SaturateOnIntegerOverflow=off  RndMeth=Floor
  log_cast_vbus : DataTypeConversion  OutDataTypeStr=single  SaturateOnIntegerOverflow=off  RndMeth=Floor
  log_cast_vleg1 : DataTypeConversion  OutDataTypeStr=single  SaturateOnIntegerOverflow=off  RndMeth=Floor
  log_cast_vlegs1 : DataTypeConversion  OutDataTypeStr=single  SaturateOnIntegerOverflow=off  RndMeth=Floor
  log_cast_vlink : DataTypeConversion  OutDataTypeStr=single  SaturateOnIntegerOverflow=off  RndMeth=Floor
  log_cast_vo : DataTypeConversion  OutDataTypeStr=single  SaturateOnIntegerOverflow=off  RndMeth=Floor
  log_cast_vs : DataTypeConversion  OutDataTypeStr=single  SaturateOnIntegerOverflow=off  RndMeth=Floor
  log_dg : ToWorkspace  VariableName=dg  SampleTime=-1
      settings: Decimation=TB.Np
  log_flags : ToWorkspace  VariableName=flags  SampleTime=-1
      settings: Decimation=TB.Np
  log_gq1 : ToWorkspace  VariableName=gq1  SampleTime=-1
      settings: Decimation=4
  log_gq2 : ToWorkspace  VariableName=gq2  SampleTime=-1
      settings: Decimation=4
  log_gs1 : ToWorkspace  VariableName=gs1  SampleTime=-1
      settings: Decimation=4
  log_gs2 : ToWorkspace  VariableName=gs2  SampleTime=-1
      settings: Decimation=4
  log_iA1 : ToWorkspace  VariableName=iA1  SampleTime=-1
  log_iA2 : ToWorkspace  VariableName=iA2  SampleTime=-1
  log_iAo : ToWorkspace  VariableName=iAo  SampleTime=-1
      settings: Decimation=4
  log_iL : ToWorkspace  VariableName=iL  SampleTime=-1
      settings: Decimation=2
  log_iLb : ToWorkspace  VariableName=iLb  SampleTime=-1
      settings: Decimation=4
  log_ibrk : ToWorkspace  VariableName=ibrk  SampleTime=-1
      settings: Decimation=2
  log_ibyp : ToWorkspace  VariableName=ibyp  SampleTime=-1
      settings: Decimation=2
  log_ih : ToWorkspace  VariableName=ih  SampleTime=-1
      settings: Decimation=2
  log_iin : ToWorkspace  VariableName=iin  SampleTime=-1
      settings: Decimation=4
  log_ilink : ToWorkspace  VariableName=ilink  SampleTime=-1
      settings: Decimation=2
  log_iload : ToWorkspace  VariableName=iload  SampleTime=-1
      settings: Decimation=4
  log_ip : ToWorkspace  VariableName=ip  SampleTime=-1
      settings: Decimation=2
  log_ir2 : ToWorkspace  VariableName=ir2  SampleTime=-1
      settings: Decimation=4
  log_ix : ToWorkspace  VariableName=ix  SampleTime=-1
      settings: Decimation=4
  log_shed : ToWorkspace  VariableName=shed  SampleTime=-1
      settings: Decimation=4
  log_st1 : ToWorkspace  VariableName=st1  SampleTime=-1
  log_st2 : ToWorkspace  VariableName=st2  SampleTime=-1
  log_sup : ToWorkspace  VariableName=sup  SampleTime=-1
      settings: Decimation=TB.Np
  log_t : ToWorkspace  VariableName=t  SampleTime=-1
      settings: Decimation=2
  log_t4 : ToWorkspace  VariableName=t4  SampleTime=-1
      settings: Decimation=4
  log_uc : ToWorkspace  VariableName=uc  SampleTime=-1
      settings: Decimation=TB.Np
  log_ucC : ToWorkspace  VariableName=ucC  SampleTime=-1
      settings: Decimation=4000
  log_vA : ToWorkspace  VariableName=vA  SampleTime=-1
      settings: Decimation=4
  log_vI : ToWorkspace  VariableName=vI  SampleTime=-1
      settings: Decimation=4
  log_vbus : ToWorkspace  VariableName=vbus  SampleTime=-1
      settings: Decimation=2
  log_vleg1 : ToWorkspace  VariableName=vleg1  SampleTime=-1
      settings: Decimation=4
  log_vlegs1 : ToWorkspace  VariableName=vlegs1  SampleTime=-1
      settings: Decimation=4
  log_vlink : ToWorkspace  VariableName=vlink  SampleTime=-1
      settings: Decimation=2
  log_vo : ToWorkspace  VariableName=vo  SampleTime=-1
      settings: Decimation=4
  log_vs : ToWorkspace  VariableName=vs  SampleTime=-1
      settings: Decimation=2
  wires:
  [iA_P1] -> Scope_StageA/1
  [iA_P2] -> Scope_StageA/2
  [vA] -> Scope_StageA/3
  [stA_shed] -> Scope_StageA/4
  [vbus] -> Scope_Bus/1
  [p_load] -> Scope_Bus/2
  [iin] -> Scope_Bus/3
  [ip] -> Scope_StageB/1
  [ih] -> Scope_StageB/2
  [ibyp] -> Scope_StageB/3
  [vs] -> Scope_StageB/4
  [vlink] -> Scope_Link/1
  [ilink] -> Scope_Link/2
  [ibrk] -> Scope_Link/3
  [iL] -> Scope_Link/4
  [r2_sup] -> Scope_State/1
  [vo] -> Scope_48V/1
  [ix] -> Scope_48V/2
  [iLb] -> Scope_48V/3
  [ir2] -> Scope_CLLC/1
  [vleg1] -> Scope_CLLC/2
  [vlegs1] -> Scope_CLLC/3
  [ctrl_dg] -> Scope_Controller/1
  [uc] -> Scope_Controller/2
  [ucC] -> Scope_Controller/3
  [t] -> log_t/1
  [vbus] -> log_cast_vbus/1
  log_cast_vbus/1 -> log_vbus/1
  [ip] -> log_cast_ip/1
  log_cast_ip/1 -> log_ip/1
  [ih] -> log_cast_ih/1
  log_cast_ih/1 -> log_ih/1
  [vs] -> log_cast_vs/1
  log_cast_vs/1 -> log_vs/1
  [vlink] -> log_cast_vlink/1
  log_cast_vlink/1 -> log_vlink/1
  [ilink] -> log_cast_ilink/1
  log_cast_ilink/1 -> log_ilink/1
  [ibyp] -> log_cast_ibyp/1
  log_cast_ibyp/1 -> log_ibyp/1
  [ibrk] -> log_cast_ibrk/1
  log_cast_ibrk/1 -> log_ibrk/1
  [iL] -> log_cast_iL/1
  log_cast_iL/1 -> log_iL/1
  [ctrl_dg] -> log_dg/1
  [uc] -> log_uc/1
  [r2_sup] -> log_sup/1
  [r2_flags] -> log_flags/1
  [iA_P1] -> log_cast_iA1/1
  log_cast_iA1/1 -> log_iA1/1
  [iA_P2] -> log_cast_iA2/1
  log_cast_iA2/1 -> log_iA2/1
  [stA_P1] -> log_cast_st1/1
  log_cast_st1/1 -> log_st1/1
  [stA_P2] -> log_cast_st2/1
  log_cast_st2/1 -> log_st2/1
  [stA_shed] -> log_cast_shed/1
  log_cast_shed/1 -> log_shed/1
  [t] -> log_t4/1
  [vA] -> log_cast_vA/1
  log_cast_vA/1 -> log_vA/1
  [iAo] -> log_cast_iAo/1
  log_cast_iAo/1 -> log_iAo/1
  [iin] -> log_cast_iin/1
  log_cast_iin/1 -> log_iin/1
  [iLb] -> log_cast_iLb/1
  log_cast_iLb/1 -> log_iLb/1
  [vI] -> log_cast_vI/1
  log_cast_vI/1 -> log_vI/1
  [vo] -> log_cast_vo/1
  log_cast_vo/1 -> log_vo/1
  [ix] -> log_cast_ix/1
  log_cast_ix/1 -> log_ix/1
  [iload] -> log_cast_iload/1
  log_cast_iload/1 -> log_iload/1
  [ir2] -> log_cast_ir2/1
  log_cast_ir2/1 -> log_ir2/1
  [vleg1] -> log_cast_vleg1/1
  log_cast_vleg1/1 -> log_vleg1/1
  [vlegs1] -> log_cast_vlegs1/1
  log_cast_vlegs1/1 -> log_vlegs1/1
  [gC_Q1] -> log_cast_gq1/1
  log_cast_gq1/1 -> log_gq1/1
  [gC_Q2] -> log_cast_gq2/1
  log_cast_gq2/1 -> log_gq2/1
  [gC_S1] -> log_cast_gs1/1
  log_cast_gs1/1 -> log_gs1/1
  [gC_S2] -> log_cast_gs2/1
  log_cast_gs2/1 -> log_gs2/1
  [ucC] -> log_ucC/1

== system TB19_R2_Integrated_Shed/S_BYP_1 ==
  note: 스위치 셀: 이상 스위치(R_on, G_off) + 역병렬 바디 다이오드(Vf, R_d)
      | 게이트: 전역 태그 "gByp" (> 0.5 이면 도통)
  D_body : fl_lib/Electrical/Electrical Elements/Diode  Vf=Vf V  Ron=Rd Ohm  Goff=Goffd 1/Ohm  i_specify=off  i_priority=None  i=0 A  i_nominal_specify=off  i_nominal_value=1  i_nominal_unit=A  v_specify=off  v_priority=None  v=0 V  v_nominal_specify=off  v_nominal_value=1  v_nominal_unit=V
  Gate_PS : nesl_utility/Simulink-PS Converter  PhysicalDomain=network_engine_domain  SubClassName=ps_input  LeftPortType=input  RightPortType=output  PseudoPeriodic=off  Frequencies=[]  NoiseDistribution=none  NoiseParameters=[]  Unit=1  AffineConversion=off  FilteringAndDerivatives=zero  SimscapeFilterOrder=1  InputFilterTimeConstant=0.001  UdotUserProvided=0
  SW : fl_lib/Electrical/Electrical Elements/Switch  R_closed=Ron Ohm  G_open=Goff 1/Ohm  Threshold=0.5  i_specify=off  i_priority=None  i=0 A  i_nominal_specify=off  i_nominal_value=1  i_nominal_unit=A  v_specify=off  v_priority=None  v=0 V  v_nominal_specify=off  v_nominal_value=1  v_nominal_unit=V
  D : PMIOPort  Side=Left
  S : PMIOPort  Port=2  Side=Right
  wires:
  [gByp] -> Gate_PS/1
  connections:
  Gate_PS/RConn1 -- SW/RConn1
  SW/LConn1 -- D/RConn1 -- D_body/RConn1
  S/RConn1 -- SW/RConn2 -- D_body/LConn1

== system TB19_R2_Integrated_Shed/S_BYP_2 ==
  note: 스위치 셀: 이상 스위치(R_on, G_off) + 역병렬 바디 다이오드(Vf, R_d)
      | 게이트: 전역 태그 "gByp" (> 0.5 이면 도통)
  D_body : fl_lib/Electrical/Electrical Elements/Diode  Vf=Vf V  Ron=Rd Ohm  Goff=Goffd 1/Ohm  i_specify=off  i_priority=None  i=0 A  i_nominal_specify=off  i_nominal_value=1  i_nominal_unit=A  v_specify=off  v_priority=None  v=0 V  v_nominal_specify=off  v_nominal_value=1  v_nominal_unit=V
  Gate_PS : nesl_utility/Simulink-PS Converter  PhysicalDomain=network_engine_domain  SubClassName=ps_input  LeftPortType=input  RightPortType=output  PseudoPeriodic=off  Frequencies=[]  NoiseDistribution=none  NoiseParameters=[]  Unit=1  AffineConversion=off  FilteringAndDerivatives=zero  SimscapeFilterOrder=1  InputFilterTimeConstant=0.001  UdotUserProvided=0
  SW : fl_lib/Electrical/Electrical Elements/Switch  R_closed=Ron Ohm  G_open=Goff 1/Ohm  Threshold=0.5  i_specify=off  i_priority=None  i=0 A  i_nominal_specify=off  i_nominal_value=1  i_nominal_unit=A  v_specify=off  v_priority=None  v=0 V  v_nominal_specify=off  v_nominal_value=1  v_nominal_unit=V
  D : PMIOPort  Side=Left
  S : PMIOPort  Port=2  Side=Right
  wires:
  [gByp] -> Gate_PS/1
  connections:
  Gate_PS/RConn1 -- SW/RConn1
  SW/LConn1 -- D/RConn1 -- D_body/RConn1
  S/RConn1 -- SW/RConn2 -- D_body/LConn1

== system TB19_R2_Integrated_Shed/StageA_Module1 ==
  note: Stage A 모듈 1: 위상 1·2 병렬(목표 정격 37.5 kW)
      | 각 위상은 영교차 추종 게이트로 자기 공진전류가 0일 때 끈다(ZCS). 두 위상은 T/4 엇갈려 시작한다.
  StageA_Phase1 : Subsystem
  StageA_Phase2 : Subsystem
  VIN : PMIOPort  Side=Left
  GND : PMIOPort  Port=2  Side=Left
  VOUT : PMIOPort  Port=3  Side=Right
  connections:
  VIN/RConn1 -- StageA_Phase1/LConn1 -- StageA_Phase2/LConn1
  GND/RConn1 -- StageA_Phase1/LConn2 -- StageA_Phase2/LConn2
  VOUT/RConn1 -- StageA_Phase1/RConn1 -- StageA_Phase2/RConn1

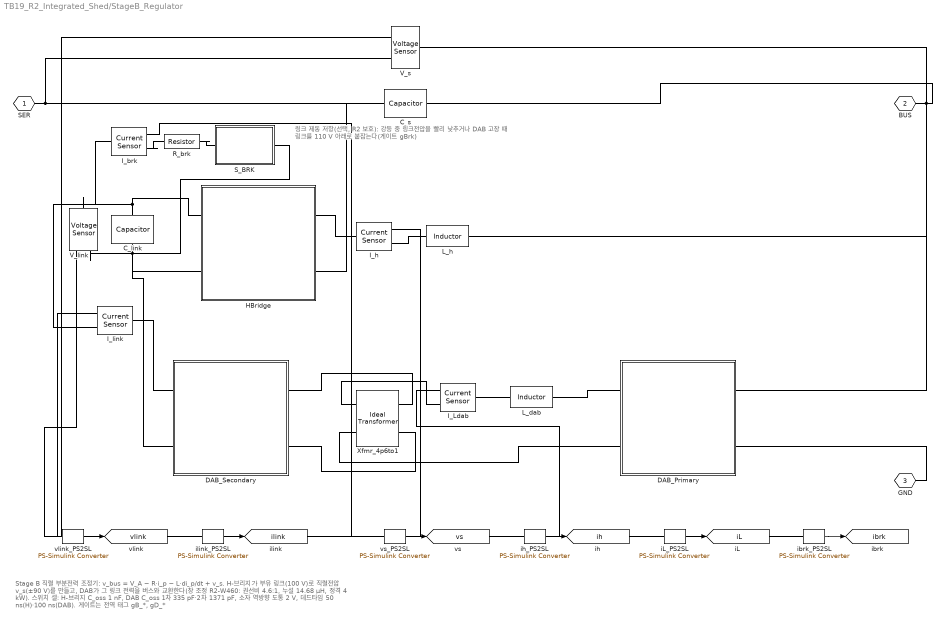
== system TB19_R2_Integrated_Shed/StageB_Regulator ==
  note: 링크 제동 저항(선택, R2 보호): 강등 중 링크전압을 빨리 낮추거나
      | DAB 고장 때 링크를 110 V 아래로 붙잡는다(게이트 gBrk)
  note: Stage B 직렬 부분전력 조정기: v_bus = V_A − R·i_p − L·di_p/dt + v_s.
      | H-브리지가 부유 링크(100 V)로 직렬전압 v_s(±90 V)를 만들고, DAB가 그 링크 전력을 버스와 교환한다(창 조정 R2-W460: 권선비 4.6:1, 누설 14.68 µH, 정격 4 kW).
      | 스위치 셀: H-브리지 C_oss 1 nF, DAB C_oss 1차 335 pF·2차 1371 pF, 소자 역방향 도통 2 V, 데드타임 50 ns(H)·100 ns(DAB). 게이트는 전역 태그 gB_*, gD_*
  C_link : fl_lib/Electrical/Electrical Elements/Capacitor  c=TB.B.Clink F  r=1e-6 Ohm  g=0 1/Ohm  i_specify=off  i_priority=None  i=0 A  i_nominal_specify=off  i_nominal_value=1  i_nominal_unit=A  v_specify=off  v_priority=None  v=0 V  v_nominal_specify=off  v_nominal_value=1  v_nominal_unit=V  vc_specify=on  vc_priority=High  vc=TB.vl0 V  vc_nominal_specify=off  vc_nominal_value=1  vc_nominal_unit=V
  C_s : fl_lib/Electrical/Electrical Elements/Capacitor  c=TB.B.Cs F  r=1e-6 Ohm  g=0 1/Ohm  i_specify=off  i_priority=None  i=0 A  i_nominal_specify=off  i_nominal_value=1  i_nominal_unit=A  v_specify=off  v_priority=None  v=0 V  v_nominal_specify=off  v_nominal_value=1  v_nominal_unit=V  vc_specify=on  vc_priority=High  vc=TB.vs0 V  vc_nominal_specify=off  vc_nominal_value=1  vc_nominal_unit=V
  DAB_Primary : Subsystem
  DAB_Secondary : Subsystem
  HBridge : Subsystem
  I_Ldab : fl_lib/Electrical/Electrical Sensors/Current Sensor
  I_brk : fl_lib/Electrical/Electrical Sensors/Current Sensor
  I_h : fl_lib/Electrical/Electrical Sensors/Current Sensor
  I_link : fl_lib/Electrical/Electrical Sensors/Current Sensor
  L_dab : fl_lib/Electrical/Electrical Elements/Inductor  l=TB.B.Ldab H  r=TB.B.Rdab Ohm  g=1e-9 1/Ohm  i_specify=off  i_priority=None  i=0 A  i_nominal_specify=off  i_nominal_value=1  i_nominal_unit=A  v_specify=off  v_priority=None  v=0 V  v_nominal_specify=off  v_nominal_value=1  v_nominal_unit=V  i_L_specify=on  i_L_priority=High  i_L=0 A  i_L_nominal_specify=off  i_L_nominal_value=1  i_L_nominal_unit=A
  L_h : fl_lib/Electrical/Electrical Elements/Inductor  l=TB.B.Lh H  r=TB.B.Rh Ohm  g=1e-9 1/Ohm  i_specify=off  i_priority=None  i=0 A  i_nominal_specify=off  i_nominal_value=1  i_nominal_unit=A  v_specify=off  v_priority=None  v=0 V  v_nominal_specify=off  v_nominal_value=1  v_nominal_unit=V  i_L_specify=on  i_L_priority=High  i_L=TB.ih0 A  i_L_nominal_specify=off  i_L_nominal_value=1  i_L_nominal_unit=A
  R_brk : fl_lib/Electrical/Electrical Elements/Resistor  R=TB.Rbrk Ohm  i_specify=off  i_priority=None  i=0 A  i_nominal_specify=off  i_nominal_value=1  i_nominal_unit=A  v_specify=off  v_priority=None  v=0 V  v_nominal_specify=off  v_nominal_value=1  v_nominal_unit=V
  S_BRK : Subsystem  mask(PRISM-Hub switch cell){Ron=TB.B.Ron, Goff=TB.B.Goff, Vf=TB.B.Vf, Rd=TB.B.Rd, Goffd=TB.B.Goffd}
      mask prompts: Ron "도통 저항 R_on [Ohm]"; Goff "차단 컨덕턴스 G_off [S]"; Vf "다이오드 순방향 전압 Vf [V]"; Rd "다이오드 도통 저항 R_d [Ohm]"; Goffd "다이오드 차단 컨덕턴스 [S]"
      mask help: 전력 반도체 스위치 셀 BRK. 게이트 태그 gBrk.
      settings: AttributesFormatString=gate: gBrk
      mask Display:
      | plot([0.05 0.35 ],[0.50 0.50 ],[0.35 0.65 ],[0.50 0.74 ],[0.65 0.95 ],[0.50 0.50 ]);
      | plot([0.20 0.20 0.42 ],[0.50 0.20 0.20 ],[0.58 0.80 0.80 ],[0.20 0.20 0.50 ]);
      | plot([0.42 0.58 0.58 0.42 ],[0.20 0.10 0.30 0.20 ],[0.42 0.42 ],[0.10 0.30 ]);
      | text(0.5,0.80,'BRK','horizontalAlignment','center','texmode','off');
      | port_label('LConn',1,'D');
      | port_label('RConn',1,'S');
  V_link : fl_lib/Electrical/Electrical Sensors/Voltage Sensor
  V_s : fl_lib/Electrical/Electrical Sensors/Voltage Sensor
  Xfmr_4p6to1 : fl_lib/Electrical/Electrical Elements/Ideal Transformer  n=TB.B.n  i1_specify=off  i1_priority=None  i1=0 A  i1_nominal_specify=off  i1_nominal_value=1  i1_nominal_unit=A  v1_specify=off  v1_priority=None  v1=0 V  v1_nominal_specify=off  v1_nominal_value=1  v1_nominal_unit=V  i2_specify=off  i2_priority=None  i2=0 A  i2_nominal_specify=off  i2_nominal_value=1  i2_nominal_unit=A  v2_specify=off  v2_priority=None  v2=0 V  v2_nominal_specify=off  v2_nominal_value=1  v2_nominal_unit=V
  iL_PS2SL : nesl_utility/PS-Simulink Converter  PhysicalDomain=network_engine_domain  SubClassName=ps_output  LeftPortType=input  RightPortType=output  PseudoPeriodic=off  Frequencies=[]  VectorFormat=inherit  Unit=inherit  AffineConversion=off
  ibrk_PS2SL : nesl_utility/PS-Simulink Converter  PhysicalDomain=network_engine_domain  SubClassName=ps_output  LeftPortType=input  RightPortType=output  PseudoPeriodic=off  Frequencies=[]  VectorFormat=inherit  Unit=inherit  AffineConversion=off
  ih_PS2SL : nesl_utility/PS-Simulink Converter  PhysicalDomain=network_engine_domain  SubClassName=ps_output  LeftPortType=input  RightPortType=output  PseudoPeriodic=off  Frequencies=[]  VectorFormat=inherit  Unit=inherit  AffineConversion=off
  ilink_PS2SL : nesl_utility/PS-Simulink Converter  PhysicalDomain=network_engine_domain  SubClassName=ps_output  LeftPortType=input  RightPortType=output  PseudoPeriodic=off  Frequencies=[]  VectorFormat=inherit  Unit=inherit  AffineConversion=off
  vlink_PS2SL : nesl_utility/PS-Simulink Converter  PhysicalDomain=network_engine_domain  SubClassName=ps_output  LeftPortType=input  RightPortType=output  PseudoPeriodic=off  Frequencies=[]  VectorFormat=inherit  Unit=inherit  AffineConversion=off
  vs_PS2SL : nesl_utility/PS-Simulink Converter  PhysicalDomain=network_engine_domain  SubClassName=ps_output  LeftPortType=input  RightPortType=output  PseudoPeriodic=off  Frequencies=[]  VectorFormat=inherit  Unit=inherit  AffineConversion=off
  SER : PMIOPort  Side=Left
  BUS : PMIOPort  Port=2  Side=Right
  GND : PMIOPort  Port=3  Side=Right
  tag scope: iL=global, ibrk=global, ih=global, ilink=global, vlink=global, vs=global
  wires:
  ibrk_PS2SL/1 -> [ibrk]
  vs_PS2SL/1 -> [vs]
  ih_PS2SL/1 -> [ih]
  vlink_PS2SL/1 -> [vlink]
  ilink_PS2SL/1 -> [ilink]
  iL_PS2SL/1 -> [iL]
  connections:
  C_s/RConn1 -- V_s/RConn2 -- SER/RConn1 -- HBridge/RConn2
  C_s/LConn1 -- V_s/LConn1 -- L_h/RConn1 -- BUS/RConn1 -- DAB_Primary/LConn1
  HBridge/RConn1 -- I_h/LConn1
  I_h/RConn2 -- L_h/LConn1
  HBridge/LConn1 -- C_link/LConn1 -- V_link/LConn1 -- I_link/RConn2 -- I_brk/LConn1
  HBridge/LConn2 -- C_link/RConn1 -- V_link/RConn2 -- DAB_Secondary/LConn2 -- S_BRK/RConn1
  DAB_Secondary/LConn1 -- I_link/LConn1
  DAB_Secondary/RConn1 -- Xfmr_4p6to1/RConn1
  DAB_Secondary/RConn2 -- Xfmr_4p6to1/RConn2
  DAB_Primary/RConn1 -- L_dab/LConn1
  L_dab/RConn1 -- I_Ldab/LConn1
  I_Ldab/RConn2 -- Xfmr_4p6to1/LConn1
  Xfmr_4p6to1/LConn2 -- DAB_Primary/RConn2
  DAB_Primary/LConn2 -- GND/RConn1
  I_brk/RConn2 -- R_brk/LConn1
  R_brk/RConn1 -- S_BRK/LConn1
  I_brk/RConn1 -- ibrk_PS2SL/LConn1
  V_s/RConn1 -- vs_PS2SL/LConn1
  I_h/RConn1 -- ih_PS2SL/LConn1
  V_link/RConn1 -- vlink_PS2SL/LConn1
  I_link/RConn1 -- ilink_PS2SL/LConn1
  I_Ldab/RConn1 -- iL_PS2SL/LConn1
